simulink model "Controller"  (R2018b)
settings: configuration reference "control_config" (kept outside this file)
values from neighbouring files (symbols this model uses):
  CONTROL_EXPORT = Simulink.Parameter(CONTROL_EXPORT_VALUE)    [controller_model_init.m]
  CONTROL_PARAM = Simulink.Parameter(CONTROL_PARAM_VALUE)    [controller_model_init.m]
undefined symbols (not defined in the file or in its folder): actuator_cmd, CONTROL_CONST, ControlMode, DiscIntNeverNeededParam, PilotMode, timestamp, VehicleStatus, VTOLState
libraries: simulink x31, FMT_Model_Lib x20
(part 2 of 3)

== system Controller/Controller/VTOL_Control_Allocation/VTOL_Control_Allocation/VTOL1/actuator_cmd_routing ==
  cmd_in : Inport
  status : Inport  Port=2
  Disarm : Subsystem
  Multiport Switch : MultiPortSwitch  DataPortForDefault=Additional data port  DiagnosticForDefault=None
  Standby : Subsystem
  cmd_out : Outport
  wires:
  Multiport Switch/1 -> cmd_out/1
  status/1 -> Multiport Switch/1
  cmd_in/1 -> Multiport Switch/4
  Disarm/1(actuator_cmd) -> Multiport Switch/5, Multiport Switch/2
  Standby/1(actuator_cmd) -> Multiport Switch/3

== system Controller/Controller/VTOL_Control_Allocation/VTOL_Control_Allocation/VTOL2/FW_Control_Allocation ==
  fw_torque_cmd : Inport
  fw_force_cmd : Inport  Port=2
  FMS_Out : Inport  Port=3
  Bias : Bias  Bias=1500
  Bias1 : Bias  Bias=CONTROL_PARAM.SERVO1_BIAS
  Bias2 : Bias  Bias=CONTROL_PARAM.SERVO2_BIAS
  Bias3 : Bias  Bias=CONTROL_PARAM.SERVO3_BIAS
  Bias4 : Bias  Bias=CONTROL_PARAM.SERVO4_BIAS
  Data Type Conversion{,1..3} (4 alike) : DataTypeConversion  OutDataTypeStr=uint16
  Demux : Demux
  FW_Effective_Matrix : Subsystem
  Gain1 : Gain  Gain=[500;500;500;500]  OutDataTypeStr=Inherit: Same as input  ParamDataTypeStr=Inherit: Same as input
  Multiply1 : Product  Multiplication=Matrix(*)  OutDataTypeStr=Inherit: Same as first input
  Mux1 : Mux  Inputs=5
  Saturation1 : Saturate  UpperLimit=up_limit  LowerLimit=lo_limit  OutDataTypeStr=uint16
  Saturation4 : Saturate  UpperLimit=1  LowerLimit=0
  Saturation5 : Saturate  UpperLimit=1  LowerLimit=-1
  Selector : Selector  InputPortWidth=3  IndexOptions=Index vector (dialog)  Indices=1  OutputSizes=1
  Signal_Select : Subsystem  Commented=on
  fw_throttle_mapping : Subsystem
  fw_actuator_cmd : Outport
  wires:
  Demux/1 -> Bias1/1
  Gain1/1 -> Bias/1
  Saturation5/1 -> Multiply1/2
  Saturation4/1 -> fw_throttle_mapping/1(thrust_cmd)
  Selector/1 -> Saturation4/1
  Demux/2 -> Bias2/1
  Demux/4 -> Bias4/1
  FW_Effective_Matrix/1(EffecMat) -> Multiply1/1
  fw_force_cmd/1 -> Selector/1
  Demux/3 -> Bias3/1
  Mux1/1 -> Saturation1/1
  Multiply1/1 -> Gain1/1
  fw_torque_cmd/1 -> Saturation5/1
  fw_throttle_mapping/1(throttle_cmd) -> Mux1/1, Signal_Select/1(throttle_cmd_in)  "main_rotor"
  FMS_Out/1 -> Signal_Select/2(FMS_Out)
  Bias/1 -> Demux/1
  Saturation1/1 -> fw_actuator_cmd/1
  Bias1/1 -> Data Type Conversion/1
  Bias2/1 -> Data Type Conversion1/1
  Bias3/1 -> Data Type Conversion2/1
  Bias4/1 -> Data Type Conversion3/1
  Data Type Conversion/1 -> Mux1/2  "aileron_left"
  Data Type Conversion1/1 -> Mux1/3  "aileron_right"
  Data Type Conversion2/1 -> Mux1/4  "tail_left"
  Data Type Conversion3/1 -> Mux1/5  "tail_right"

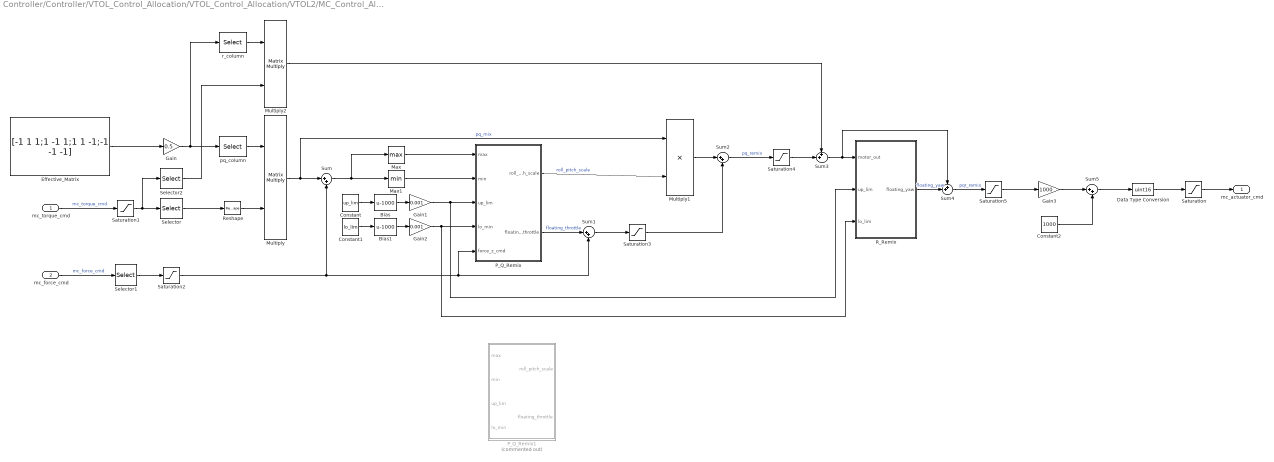
== system Controller/Controller/VTOL_Control_Allocation/VTOL_Control_Allocation/VTOL2/MC_Control_Allocation ==
  mc_torque_cmd : Inport
  mc_force_cmd : Inport  Port=2
  Bias : Bias  Bias=-1000
  Bias1 : Bias  Bias=-1000
  Constant : Constant  Value=up_lim  OutDataTypeStr=single
  Constant1 : Constant  Value=lo_lim  OutDataTypeStr=single
  Constant2 : Constant  Value=1000  OutDataTypeStr=uint32
  Data Type Conversion : DataTypeConversion  OutDataTypeStr=uint16
  Effective_Matrix : Constant  Value=[-1 1 1;1 -1 1;1 1 -1;-1 -1 -1]  OutDataTypeStr=single
  Gain : Gain  Gain=0.5
  Gain1 : Gain  Gain=0.001
  Gain2 : Gain  Gain=0.001
  Gain3 : Gain  Gain=1000  OutDataTypeStr=uint32
  Max : MinMax  Function=max
  Max1 : MinMax
  Multiply : Product  Multiplication=Matrix(*)  OutDataTypeStr=single
  Multiply1 : Product  OutDataTypeStr=single
  Multiply2 : Product  Multiplication=Matrix(*)  OutDataTypeStr=single
  P_Q_Remix : Subsystem
  P_Q_Remix1 : Subsystem  Commented=on
  R_Remix : MATLAB Function  TreatAsAtomicUnit=on
  Reshape : Reshape  OutputDimensionality=Column vector (2-D)
  Saturation : Saturate  UpperLimit=up_lim  LowerLimit=lo_lim
  Saturation1 : Saturate  UpperLimit=1  LowerLimit=-1
  Saturation{2..5} (4 alike) : Saturate  UpperLimit=1  LowerLimit=0
  Selector : Selector  InputPortWidth=3  IndexOptions=Index vector (dialog)  Indices=[1 2]  OutputSizes=1
  Selector1 : Selector  InputPortWidth=3  IndexOptions=Index vector (dialog)  Indices=3  OutputSizes=1
  Selector2 : Selector  InputPortWidth=3  IndexOptions=Index vector (dialog)  Indices=3  OutputSizes=1
  Sum{,1..2,5} (4 alike) : Sum  Inputs=|++
  Sum3 : Sum  Inputs=++|
  Sum4 : Sum  Inputs=++|
  pq_column : Selector  NumberOfDimensions=2  InputPortWidth=3  IndexOptions=Index vector (dialog),Index vector (dialog)  Indices=[1:4],[1 2]  OutputSizes=1,1
  r_column : Selector  NumberOfDimensions=2  InputPortWidth=3  IndexOptions=Index vector (dialog),Index vector (dialog)  Indices=[1:4],3  OutputSizes=1,1
  mc_actuator_cmd : Outport
  wires:
  Multiply/1 -> Multiply1/1, Sum/1  "pq_mix"
  Effective_Matrix/1 -> Gain/1
  mc_force_cmd/1 -> Selector1/1  "mc_force_cmd"
  Sum/1 -> Max/1, Max1/1
  Saturation/1 -> mc_actuator_cmd/1
  Reshape/1 -> Multiply/2
  Selector/1 -> Reshape/1
  Saturation1/1 -> Selector2/1, Selector/1
  Selector1/1 -> Saturation2/1
  pq_column/1 -> Multiply/1
  Max/1 -> P_Q_Remix/1(max)
  Max1/1 -> P_Q_Remix/2(min)
  Gain/1 -> r_column/1, pq_column/1
  P_Q_Remix/2(floating_throttle) -> Sum1/1  "floating_throttle"
  P_Q_Remix/1(roll_pitch_scale) -> Multiply1/2  "roll_pitch_scale"
  Multiply1/1 -> Sum2/1
  Sum1/1 -> Saturation3/1
  Sum2/1 -> Saturation4/1  "pq_remix"
  r_column/1 -> Multiply2/1
  Selector2/1 -> Multiply2/2
  Multiply2/1 -> Sum3/1
  Saturation4/1 -> Sum3/2
  Sum3/1 -> Sum4/1, R_Remix/1(motor_out)
  Constant/1 -> Bias/1
  Constant1/1 -> Bias1/1
  R_Remix/1(floating_yaw) -> Sum4/2  "floating_yaw"
  Sum4/1 -> Saturation5/1  "pqr_remix"
  Data Type Conversion/1 -> Saturation/1
  Bias/1 -> Gain1/1
  Gain1/1 -> R_Remix/2(up_lim), P_Q_Remix/3(up_lim)
  Bias1/1 -> Gain2/1
  Gain2/1 -> R_Remix/3(lo_lim), P_Q_Remix/4(lo_min)
  mc_torque_cmd/1 -> Saturation1/1  "mc_torque_cmd"
  Sum5/1 -> Data Type Conversion/1
  Saturation5/1 -> Gain3/1
  Gain3/1 -> Sum5/1
  Constant2/1 -> Sum5/2
  Saturation2/1 -> Sum1/2, P_Q_Remix/5(force_z_cmd), Sum/2
  Saturation3/1 -> Sum2/2

== system Controller/Controller/VTOL_Control_Allocation/VTOL_Control_Allocation/VTOL2/actuator_cmd_routing ==
  cmd_in : Inport
  status : Inport  Port=2
  Disarm : Subsystem
  Multiport Switch : MultiPortSwitch  DataPortForDefault=Additional data port  DiagnosticForDefault=None
  Standby : Subsystem
  cmd_out : Outport
  wires:
  Multiport Switch/1 -> cmd_out/1
  Standby/1(actuator_cmd) -> Multiport Switch/3
  status/1 -> Multiport Switch/1
  cmd_in/1 -> Multiport Switch/4
  Disarm/1(actuator_cmd) -> Multiport Switch/5, Multiport Switch/2

== system Controller/Controller/FW_Controller/FW_Controller/Attitude_Control/Innerloop_Rate_Control/PI_Control ==
  error : Inport
  reset : Inport  Port=2
  Add1 : Sum
  I_Control : Subsystem  mask{p_ki=CONTROL_PARAM.FW_ROLL_RATE_I, q_ki=CONTROL_PARAM.FW_PITCH_RATE_I, r_ki=CONTROL_PARAM.FW_YAW_RATE_I, max_i=CONTROL_PARAM.FW_RATE_I_MAX, min_i=CONTROL_PARAM.FW_RATE_I_MIN}
  P_Control : Subsystem  mask{p_kp=CONTROL_PARAM.FW_ROLL_RATE_P, q_kp=CONTROL_PARAM.FW_PITCH_RATE_P, r_kp=CONTROL_PARAM.FW_YAW_RATE_P}
  pi_out : Outport
  wires:
  Add1/1 -> pi_out/1
  I_Control/1(i_out) -> Add1/2  "fw_i_out"
  error/1 -> P_Control/1(err), I_Control/1(err)
  P_Control/1(p_out) -> Add1/1  "fw_p_out"
  reset/1 -> I_Control/2(reset)

== system Controller/Controller/FW_Controller/FW_Controller/Attitude_Control/Innerloop_Rate_Control/PI_scaler ==
  VT : Inport
  Divide : Product  Inputs=*/
  First Order LPF : FMT_Model_Lib/Filter/First Order LPF  fc=5
      settings: SourceProductName=FMT Toolbox
  Saturation : Saturate  UpperLimit=1  LowerLimit=0
  Square : Math  Operator=square  SaturateOnIntegerOverflow=on
  Square1 : Math  Operator=square  SaturateOnIntegerOverflow=on
  trim_speed : Constant  Value=CONTROL_PARAM.FW_AIRSPEED_TRIM
  PI_scale : Outport
  wires:
  Square1/1 -> Divide/2
  trim_speed/1 -> Square/1
  Square/1 -> Divide/1
  VT/1 -> Square1/1
  Saturation/1 -> First Order LPF/1
  Divide/1 -> Saturation/1
  First Order LPF/1 -> PI_scale/1

== system Controller/Controller/FW_Controller/FW_Controller/Attitude_Control/Innerloop_Rate_Control/VT_scaler ==
  VT : Inport
  Divide : Product  Inputs=*/
  First Order LPF : FMT_Model_Lib/Filter/First Order LPF  fc=5
      settings: SourceProductName=FMT Toolbox
  Saturation : Saturate  UpperLimit=1  LowerLimit=0
  trim_speed : Constant  Value=CONTROL_PARAM.FW_AIRSPEED_TRIM
  FF_scale : Outport
  wires:
  trim_speed/1 -> Divide/1
  VT/1 -> Divide/2
  Saturation/1 -> First Order LPF/1
  Divide/1 -> Saturation/1
  First Order LPF/1 -> FF_scale/1

== system Controller/Controller/FW_Controller/FW_Controller/Attitude_Control/Outloop_Angle_Control/Attitude_Controller ==
  att_cmd : Inport
  INS_Out : Inport  Port=2
  Error : Subsystem
  P_Controller : Subsystem
  phi_theta_rate_cmd : Outport
  wires:
  INS_Out/1 -> Error/2(INS_Out)
  P_Controller/1(u) -> phi_theta_rate_cmd/1
  att_cmd/1 -> Error/1(att_cmd)
  Error/1(euler_err_rad) -> P_Controller/1(error)

== system Controller/Controller/FW_Controller/FW_Controller/Attitude_Control/Outloop_Angle_Control/Heading_Controller ==
  fw_att_cmd : Inport
  FMS_Out : Inport  Port=2
  VT : Inport  Port=3
  Bus Selector2 : BusSelector  OutputSignals=psi_rate_cmd
  Demux : Demux  Outputs=2
  Saturation : Saturate  UpperLimit=CONTROL_PARAM.FW_R_CMD_LIM  LowerLimit=-CONTROL_PARAM.FW_R_CMD_LIM
  Sum : Sum  Inputs=++|
  Turning_Coordination : Subsystem
  psi_rate_cmd : Outport
  wires:
  Turning_Coordination/1(psi_rate_sp) -> Sum/2  "fw_psi_rate_sp"
  Sum/1 -> Saturation/1
  FMS_Out/1 -> Bus Selector2/1
  VT/1 -> Turning_Coordination/3(VT)
  Bus Selector2/1 -> Sum/1  "<psi_rate_cmd>"
  fw_att_cmd/1 -> Demux/1
  Demux/1 -> Turning_Coordination/1(phi_sp)
  Demux/2 -> Turning_Coordination/2(theta_sp)
  Saturation/1 -> psi_rate_cmd/1

== system Controller/Controller/FW_Controller/FW_Controller/Attitude_Control/Outloop_Angle_Control/Signal_Select ==
  att_cmd_rad : Inport
  FMS_Out : Inport  Port=2
  Bus Selector : BusSelector  OutputSignals=ctrl_mode
  Bus Selector1 : BusSelector  OutputSignals=phi_cmd
  Bus Selector2 : BusSelector  OutputSignals=ctrl_mode
  Bus Selector3 : BusSelector  OutputSignals=theta_cmd
  Compare To Constant : simulink/Logic and Bit Operations/Compare To Constant  relop===  const=uint8([ControlMode.Stabilize, ControlMode.ALTCTL])  OutDataTypeStr=boolean
  Compare To Constant1 : simulink/Logic and Bit Operations/Compare To Constant  relop===  const=uint8([ControlMode.Stabilize])  OutDataTypeStr=boolean
  Logical Operator : Logic  Operator=OR  Inputs=1  AllPortsSameDT=off  OutDataTypeStr=boolean
  Logical Operator1 : Logic  Operator=OR  Inputs=1  AllPortsSameDT=off  OutDataTypeStr=boolean
  Mux : Mux  Inputs=2
  Selector : Selector  InputPortWidth=2  IndexOptions=Index vector (dialog)  Indices=1  OutputSizes=1
  Selector1 : Selector  InputPortWidth=2  IndexOptions=Index vector (dialog)  Indices=2  OutputSizes=1
  Switch : Switch  Criteria=u2 > Threshold
  Switch1 : Switch  Criteria=u2 > Threshold
  fw_att_cmd : Outport
  wires:
  Compare To Constant/1 -> Logical Operator/1
  att_cmd_rad/1 -> Selector/1, Selector1/1
  Bus Selector/1 -> Compare To Constant/1  "<ctrl_mode>"
  FMS_Out/1 -> Bus Selector2/1, Bus Selector3/1, Bus Selector1/1, Bus Selector/1
  Bus Selector1/1 -> Switch/1  "<phi_cmd>"
  Logical Operator/1 -> Switch/2
  Selector/1 -> Switch/3
  Logical Operator1/1 -> Switch1/2
  Compare To Constant1/1 -> Logical Operator1/1
  Bus Selector2/1 -> Compare To Constant1/1  "<ctrl_mode>"
  Bus Selector3/1 -> Switch1/1  "<theta_cmd>"
  Selector1/1 -> Switch1/3
  Switch/1 -> Mux/1  "phi_cmd"
  Switch1/1 -> Mux/2  "theta_cmd"
  Mux/1 -> fw_att_cmd/1

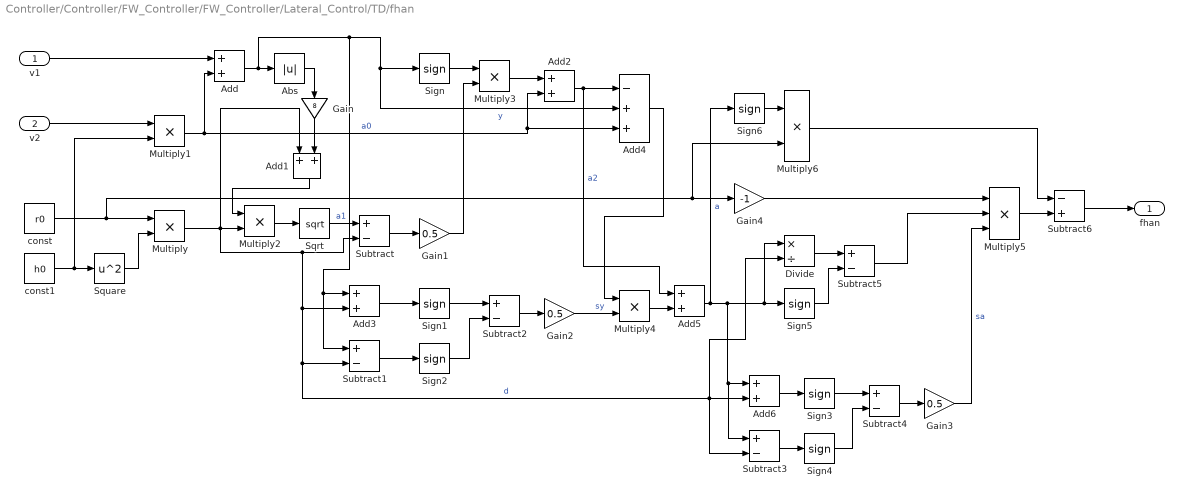
== system Controller/Controller/FW_Controller/FW_Controller/Lateral_Control/TD/fhan  ==
  v1 : Inport
  v2 : Inport  Port=2
  Abs : Abs
  Add{,1..3,5..6} (6 alike) : Sum  OutDataTypeStr=Inherit: Same as first input
  Add4 : Sum  Inputs=-++
  Divide : Product  Inputs=*/
  Gain : Gain  Gain=8
  Gain1 : Gain  Gain=0.5  OutDataTypeStr=Inherit: Same as input
  Gain2 : Gain  Gain=0.5  OutDataTypeStr=Inherit: Same as input
  Gain3 : Gain  Gain=0.5  OutDataTypeStr=Inherit: Same as input
  Gain4 : Gain  Gain=-1  OutDataTypeStr=Inherit: Same as input
  Multiply{,1..3} (4 alike) : Product  OutDataTypeStr=Inherit: Same as first input
  Multiply4 : Product  OutDataTypeStr=single
  Multiply5 : Product  Inputs=3
  Multiply6 : Product  OutDataTypeStr=single
  Sign{,1..6} (7 alike) : Signum
  Sqrt : Sqrt  SaturateOnIntegerOverflow=on
  Square : Math  Operator=square  SaturateOnIntegerOverflow=on
  Subtract{,1..5} (6 alike) : Sum  Inputs=+-  OutDataTypeStr=Inherit: Same as first input
  Subtract6 : Sum  Inputs=-+  OutDataTypeStr=Inherit: Same as first input
  const : Constant  Value=r0  OutDataTypeStr=single
  const1 : Constant  Value=h0  OutDataTypeStr=single
  fhan : Outport
  wires:
  v1/1 -> Add/1
  Sign/1 -> Multiply3/1
  Gain2/1 -> Multiply4/2  "sy"
  v2/1 -> Multiply1/1
  Gain3/1 -> Multiply5/3  "sa"
  Subtract/1 -> Gain1/1
  Subtract6/1 -> fhan/1
  Sign2/1 -> Subtract2/2
  Sign4/1 -> Subtract4/2
  Abs/1 -> Gain/1
  Add4/1 -> Multiply4/1
  Sign5/1 -> Subtract5/2
  Sqrt/1 -> Subtract/1  "a1"
  Subtract3/1 -> Sign4/1
  Add1/1 -> Multiply2/1
  Subtract1/1 -> Sign2/1
  Divide/1 -> Subtract5/1
  Multiply3/1 -> Add2/1
  Gain/1 -> Add1/2
  const/1 -> Multiply6/2, Gain4/1, Multiply/1
  Add3/1 -> Sign1/1
  Subtract5/1 -> Multiply5/2
  Multiply4/1 -> Add5/2
  const1/1 -> Multiply1/2, Square/1
  Add5/1 -> Sign6/1, Sign5/1, Divide/1, Subtract3/1, Add6/1  "a"
  Multiply1/1 -> Add4/3, Add2/2, Add/2  "a0"
  Add/1 -> Subtract1/1, Add3/1, Add4/2, Sign/1, Abs/1  "y"
  Subtract2/1 -> Gain2/1
  Add2/1 -> Add4/1, Add5/1  "a2"
  Subtract4/1 -> Gain3/1
  Gain4/1 -> Multiply5/1
  Multiply5/1 -> Subtract6/2
  Sign6/1 -> Multiply6/1
  Sign3/1 -> Subtract4/1
  Add6/1 -> Sign3/1
  Multiply/1 -> Subtract/2, Divide/2, Subtract3/2, Add6/2, Subtract1/2, Add3/2, Add1/1, Multiply2/2  "d"
  Multiply6/1 -> Subtract6/1
  Gain1/1 -> Multiply3/2
  Square/1 -> Multiply/2
  Multiply2/1 -> Sqrt/1
  Sign1/1 -> Subtract2/1

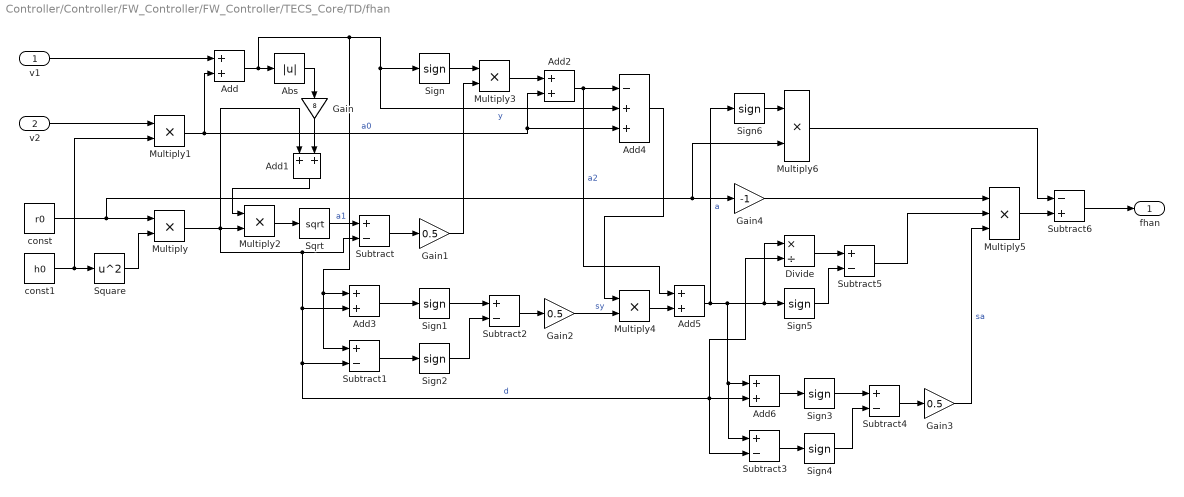
== system Controller/Controller/FW_Controller/FW_Controller/TECS_Core/TD/fhan  ==
  v1 : Inport
  v2 : Inport  Port=2
  Abs : Abs
  Add{,1..3,5..6} (6 alike) : Sum  OutDataTypeStr=Inherit: Same as first input
  Add4 : Sum  Inputs=-++
  Divide : Product  Inputs=*/
  Gain : Gain  Gain=8
  Gain1 : Gain  Gain=0.5  OutDataTypeStr=Inherit: Same as input
  Gain2 : Gain  Gain=0.5  OutDataTypeStr=Inherit: Same as input
  Gain3 : Gain  Gain=0.5  OutDataTypeStr=Inherit: Same as input
  Gain4 : Gain  Gain=-1  OutDataTypeStr=Inherit: Same as input
  Multiply{,1..3} (4 alike) : Product  OutDataTypeStr=Inherit: Same as first input
  Multiply4 : Product  OutDataTypeStr=single
  Multiply5 : Product  Inputs=3
  Multiply6 : Product  OutDataTypeStr=single
  Sign{,1..6} (7 alike) : Signum
  Sqrt : Sqrt  SaturateOnIntegerOverflow=on
  Square : Math  Operator=square  SaturateOnIntegerOverflow=on
  Subtract{,1..5} (6 alike) : Sum  Inputs=+-  OutDataTypeStr=Inherit: Same as first input
  Subtract6 : Sum  Inputs=-+  OutDataTypeStr=Inherit: Same as first input
  const : Constant  Value=r0  OutDataTypeStr=single
  const1 : Constant  Value=h0  OutDataTypeStr=single
  fhan : Outport
  wires:
  v1/1 -> Add/1
  Sign/1 -> Multiply3/1
  Gain2/1 -> Multiply4/2  "sy"
  v2/1 -> Multiply1/1
  Gain3/1 -> Multiply5/3  "sa"
  Subtract/1 -> Gain1/1
  Subtract6/1 -> fhan/1
  Sign2/1 -> Subtract2/2
  Sign4/1 -> Subtract4/2
  Abs/1 -> Gain/1
  Add4/1 -> Multiply4/1
  Sign5/1 -> Subtract5/2
  Sqrt/1 -> Subtract/1  "a1"
  Subtract3/1 -> Sign4/1
  Add1/1 -> Multiply2/1
  Subtract1/1 -> Sign2/1
  Divide/1 -> Subtract5/1
  Multiply3/1 -> Add2/1
  Gain/1 -> Add1/2
  const/1 -> Multiply6/2, Gain4/1, Multiply/1
  Add3/1 -> Sign1/1
  Subtract5/1 -> Multiply5/2
  Multiply4/1 -> Add5/2
  const1/1 -> Multiply1/2, Square/1
  Add5/1 -> Sign6/1, Sign5/1, Divide/1, Subtract3/1, Add6/1  "a"
  Multiply1/1 -> Add4/3, Add2/2, Add/2  "a0"
  Add/1 -> Subtract1/1, Add3/1, Add4/2, Sign/1, Abs/1  "y"
  Subtract2/1 -> Gain2/1
  Add2/1 -> Add4/1, Add5/1  "a2"
  Subtract4/1 -> Gain3/1
  Gain4/1 -> Multiply5/1
  Multiply5/1 -> Subtract6/2
  Sign6/1 -> Multiply6/1
  Sign3/1 -> Subtract4/1
  Add6/1 -> Sign3/1
  Multiply/1 -> Subtract/2, Divide/2, Subtract3/2, Add6/2, Subtract1/2, Add3/2, Add1/1, Multiply2/2  "d"
  Multiply6/1 -> Subtract6/1
  Gain1/1 -> Multiply3/2
  Square/1 -> Multiply/2
  Multiply2/1 -> Sqrt/1
  Sign1/1 -> Subtract2/1

== system Controller/Controller/FW_Controller/FW_Controller/TECS_Core/path_angle_control/Flight_Path_Angle ==
  INS_Out : Inport
  gamma_dir : Inport  Port=2
  speed : Inport  Port=3
  Asin : Trigonometry  Operator=atan
  Bus Selector2 : BusSelector  OutputSignals=vd
  Dead Zone : DeadZone  LowerValue=-0.1  UpperValue=0.1  SaturateOnIntegerOverflow=on
  Divide : Product  Inputs=/*
  Gain : Gain  Gain=-1
  Multiply1 : Product
  Saturation1 : Saturate  UpperLimit=pi/4  LowerLimit=-pi/4
  gamma : Outport
  wires:
  INS_Out/1 -> Bus Selector2/1
  Gain/1 -> Divide/2
  Divide/1 -> Asin/1
  Bus Selector2/1 -> Dead Zone/1  "<vd>"
  Asin/1 -> Multiply1/2
  speed/1 -> Divide/1
  Saturation1/1 -> gamma/1
  Dead Zone/1 -> Gain/1
  Multiply1/1 -> Saturation1/1
  gamma_dir/1 -> Multiply1/1

== system Controller/Controller/FW_Controller/FW_Controller/TECS_Core/path_angle_control/Fly_Speed ==
  INS_Out : Inport
  Bitwise AND : simulink/Logic and Bit Operations/Bitwise Operator  logicop=AND  UseBitMask=on  BitMask=bin2dec('10000')  BitMaskRealWorld=Stored Integer
  Bus Selector1 : BusSelector  OutputSignals=flag,airspeed
  Bus Selector2 : BusSelector  OutputSignals=vn,ve,vd
  Bus Selector3 : BusSelector  OutputSignals=quat
  Multiply : Product  Multiplication=Matrix(*)
  Mux : Mux  Inputs=3
  Quaternion To DCM : FMT_Model_Lib/Quaternion/Quaternion To DCM
      settings: SourceProductName=FMT Toolbox
  Saturation : Saturate  UpperLimit=100  LowerLimit=8
  Selector : Selector  InputPortWidth=3  IndexOptions=Index vector (dialog)  Indices=1  OutputSizes=1
  Switch : Switch  Criteria=u2 > Threshold
  speed : Outport
  wires:
  Bus Selector3/1 -> Quaternion To DCM/1  "<quat>"
  Multiply/1 -> Selector/1
  Bus Selector2/3 -> Mux/3  "<vd>"
  Mux/1 -> Multiply/2
  Quaternion To DCM/1 -> Multiply/1
  Bus Selector2/2 -> Mux/2  "<ve>"
  Bus Selector2/1 -> Mux/1  "<vn>"
  Bus Selector1/2 -> Switch/3  "<airspeed>"
  Bus Selector1/1 -> Bitwise AND/1  "<flag>"
  Bitwise AND/1 -> Switch/2
  INS_Out/1 -> Bus Selector3/1, Bus Selector1/1, Bus Selector2/1
  Selector/1 -> Switch/1
  Switch/1 -> Saturation/1
  Saturation/1 -> speed/1

== system Controller/Controller/FW_Controller/FW_Controller/TECS_Core/path_angle_control/Subsystem ==
  INS_Out : Inport
  Bitwise AND : simulink/Logic and Bit Operations/Bitwise Operator  logicop=AND  UseBitMask=on  BitMask=bin2dec('10000')  BitMaskRealWorld=Stored Integer
  Bus Selector1 : BusSelector  OutputSignals=flag
  Bus Selector2 : BusSelector  OutputSignals=vn,ve,vd
  Bus Selector3 : BusSelector  OutputSignals=psi
  Constant : Constant  OutDataTypeStr=single
  Dead Zone : DeadZone  LowerValue=-1  UpperValue=1  SaturateOnIntegerOverflow=on
  Multiply : Product  Multiplication=Matrix(*)
  Mux : Mux  Inputs=3
  Psi To DCM : FMT_Model_Lib/Transformation/Psi To DCM
      settings: SourceProductName=FMT Toolbox
  Selector : Selector  InputPortWidth=3  IndexOptions=Index vector (dialog)  Indices=1  OutputSizes=1
  Sign : Signum
  Switch : Switch  Criteria=u2 > Threshold
  gamma_dir : Outport
  wires:
  Psi To DCM/1 -> Multiply/1
  Bus Selector2/3 -> Mux/3  "<vd>"
  Selector/1 -> Dead Zone/1
  Bus Selector2/2 -> Mux/2  "<ve>"
  Bus Selector3/1 -> Psi To DCM/1  "<psi>"
  Multiply/1 -> Selector/1
  Dead Zone/1 -> Sign/1
  Bus Selector2/1 -> Mux/1  "<vn>"
  Mux/1 -> Multiply/2
  INS_Out/1 -> Bus Selector1/1, Bus Selector2/1, Bus Selector3/1
  Sign/1 -> Switch/1
  Bus Selector1/1 -> Bitwise AND/1  "<flag>"
  Bitwise AND/1 -> Switch/2
  Switch/1 -> gamma_dir/1
  Constant/1 -> Switch/3

== system Controller/Controller/FW_Controller/FW_Controller/TECS_Core/path_angle_control/Target_Flight_Path_Angle ==
  FMS_Out : Inport
  gamma_dir : Inport  Port=2
  speed : Inport  Port=3
  Asin : Trigonometry  Operator=atan
  Bus Selector : BusSelector  OutputSignals=w_cmd
  Divide : Product  Inputs=*/
  Gain : Gain  Gain=-1
  Multiply1 : Product
  Saturation2 : Saturate  UpperLimit=pi/4  LowerLimit=-pi/4
  gamma_sp : Outport
  wires:
  FMS_Out/1 -> Bus Selector/1
  Bus Selector/1 -> Gain/1  "<w_cmd>"
  Divide/1 -> Asin/1
  Gain/1 -> Divide/1
  speed/1 -> Divide/2
  Saturation2/1 -> gamma_sp/1
  Asin/1 -> Multiply1/1
  Multiply1/1 -> Saturation2/1
  gamma_dir/1 -> Multiply1/2

== system Controller/Controller/FW_Controller/FW_Controller/TECS_Core/pitch_controller/D_control ==
  err : Inport
  reset : Inport  Port=2
  DT Filter : FMT_Model_Lib/Filter/DT Filter  fc=10
      settings: SourceProductName=FMT Toolbox
  Gain : Gain  Gain=CONTROL_PARAM.FW_TECS_PITCH_D
  d_out : Outport
  wires:
  reset/1 -> DT Filter/2
  DT Filter/1 -> Gain/1
  Gain/1 -> d_out/1
  err/1 -> DT Filter/1

== system Controller/Controller/FW_Controller/FW_Controller/TECS_Core/pitch_controller/I_control ==
  err : Inport
  reset : Inport  Port=2
  " " : DiscreteIntegrator  ExternalReset=level  InitialConditionSource=external  SampleTime=-1  LimitOutput=on  UpperSaturationLimit=CONTROL_PARAM.FW_TECS_PITCH_I_LIM  LowerSaturationLimit=-CONTROL_PARAM.FW_TECS_PITCH_I_LIM  ICPrevOutput=DiscIntNeverNeededParam  ICPrevScaledInput=DiscIntNeverNeededParam
  Gain3 : Gain  Gain=CONTROL_PARAM.FW_TECS_PITCH_I
  Zero1 : Constant  Value=0  OutDataTypeStr=Inherit: Inherit via back propagation
  i_out : Outport
  wires:
  Zero1/1 -> " "/3
  " "/1 -> i_out/1
  Gain3/1 -> " "/1
  err/1 -> Gain3/1
  reset/1 -> " "/2

== system Controller/Controller/MC_Controller/Horizontal_Control/Attitude_Controller/Inner_Loop/ATT_Cmd_Mixer ==
  FMS_Out : Inport
  euler_rate_cmd : Inport  Port=2
  aux_mc_cmd : Inport  Port=3
  INS_Out : Inport  Port=4
  Backward_Mixer : Subsystem  mask{max=8, min=2}
  Bus Selector1 : BusSelector  OutputSignals=ext_state
  Bus Selector2 : BusSelector  OutputSignals=psi_rate_cmd
  Bus Selector3 : BusSelector  OutputSignals=phi,theta
  Demux : Demux  Outputs=3
  Euler To Angle Rate : FMT_Model_Lib/Math/Euler To Angle Rate
      settings: SourceProductName=FMT Toolbox
  Fly_Speed : Subsystem
  Forward_Mixer : Subsystem  mask{max=8, min=2}
  Multiport Switch : MultiPortSwitch  DataPortOrder=Specify indices  DataPortIndices={uint8(VTOLState.ForwardTrans),uint8(VTOLState.BackwardTrans),uint8(VTOLState.Fixwing),uint8(VTOLState.Stall),uint8(VTOLState.Multicopter)}  DiagnosticForDefault=None
  Mux : Mux  Inputs=3
  Mux1 : Mux  Inputs=2
  Mux2 : Mux  Inputs=2
  Saturation : Saturate  UpperLimit=CONTROL_PARAM.MC_R_CMD_LIM  LowerLimit=-CONTROL_PARAM.MC_R_CMD_LIM
  Saturation1 : Saturate  UpperLimit=CONTROL_PARAM.MC_P_Q_CMD_LIM  LowerLimit=-CONTROL_PARAM.MC_P_Q_CMD_LIM
  Saturation2 : Saturate  UpperLimit=CONTROL_PARAM.MC_P_Q_CMD_LIM  LowerLimit=-CONTROL_PARAM.MC_P_Q_CMD_LIM
  rate_cmd_radPs : Outport
  wires:
  Bus Selector3/1 -> Mux2/1  "<phi>"
  Mux2/1 -> Euler To Angle Rate/1
  Bus Selector3/2 -> Mux2/2  "<theta>"
  Bus Selector2/1 -> Mux1/2  "<psi_rate_cmd>"
  FMS_Out/1 -> Bus Selector2/1, Bus Selector1/1
  INS_Out/1 -> Fly_Speed/1(INS_Out), Bus Selector3/1
  Euler To Angle Rate/1 -> Demux/1  "ang_rate"
  euler_rate_cmd/1 -> Mux1/1
  Demux/1 -> Saturation1/1
  Demux/2 -> Saturation2/1
  Demux/3 -> Saturation/1
  Saturation1/1 -> Mux/1
  Mux/1 -> rate_cmd_radPs/1
  Saturation2/1 -> Mux/2
  Saturation/1 -> Mux/3
  Bus Selector1/1 -> Multiport Switch/1  "<ext_state>"
  Multiport Switch/1 -> Euler To Angle Rate/2  "euler_rate"
  aux_mc_cmd/1 -> Multiport Switch/5, Multiport Switch/4, Forward_Mixer/2(aux_cmd), Backward_Mixer/2(aux_cmd)  "aux_rate_cmd"
  Backward_Mixer/1(mix_rate_cmd) -> Multiport Switch/3
  Forward_Mixer/1(mix_rate_cmd) -> Multiport Switch/2
  Mux1/1 -> Forward_Mixer/1(mc_cmd), Backward_Mixer/1(mc_cmd), Multiport Switch/6  "mc_rate_cmd"
  Fly_Speed/1(speed) -> Backward_Mixer/3(VT), Forward_Mixer/3(VT)

== system Controller/Controller/MC_Controller/Horizontal_Control/Attitude_Controller/Inner_Loop/Rate_Controller ==
  rate_cmd_radPs : Inport
  INS_Out : Inport  Port=2
  reset : Inport  Port=3
  Error : Subsystem
  Feedforward_Controller : Subsystem
  PID_Controller : Subsystem
  Sum : Sum  Inputs=++|
  rate_dot_cmd_B : Outport
  wires:
  INS_Out/1 -> Error/2(INS_Out)
  Error/1(rate_err_radPs) -> PID_Controller/1(rate_err_radPs)
  rate_cmd_radPs/1 -> Feedforward_Controller/1(rate_cmd_radPs), Error/1(rate_cmd_radPs)  "yy1"
  reset/1 -> PID_Controller/2(reset)
  PID_Controller/1(rate_dot_cmd_B) -> Sum/2
  Feedforward_Controller/1(rate_dot_cmd_B) -> Sum/1
  Sum/1 -> rate_dot_cmd_B/1

== system Controller/Controller/MC_Controller/Horizontal_Control/Attitude_Controller/Outter_Loop/Attitude_Controller ==
  att_cmd_rad : Inport
  INS_Out : Inport  Port=2
  Error : Subsystem
  Sqrt_Root_Controller : Subsystem
  euler_rate_cmd_radPs : Outport
  wires:
  INS_Out/1 -> Error/2(INS_Out)
  Sqrt_Root_Controller/1(euler_rate_cmd_radPs) -> euler_rate_cmd_radPs/1
  att_cmd_rad/1 -> Error/1(att_cmd)
  Error/1(euler_err_rad) -> Sqrt_Root_Controller/1(euler_err_rad)

== system Controller/Controller/MC_Controller/Horizontal_Control/Attitude_Controller/Outter_Loop/Signal_Select ==
  note: mode:
      | 0: Unknown
      | 1: Mission
      | 2: Position
      | 3: Altitude Hold
      | 4: Manual Mode
      | 5: Acro Mode
      | 6: Offboard
  att_cmd_rad : Inport
  FMS_Out : Inport  Port=2
  Bus Selector : BusSelector  OutputSignals=ctrl_mode
  Bus Selector1 : BusSelector  OutputSignals=phi_cmd,theta_cmd
  Compare To Constant : simulink/Logic and Bit Operations/Compare To Constant  relop===  const=uint8([ControlMode.Stabilize, ControlMode.ALTCTL])  OutDataTypeStr=boolean
  Compare To Constant1 : simulink/Logic and Bit Operations/Compare To Constant  relop===  const=uint8(ControlMode.Offboard)  OutDataTypeStr=boolean
  Logical Operator : Logic  Operator=OR  Inputs=1  AllPortsSameDT=off  OutDataTypeStr=boolean
  Mux : Mux  Inputs=2
  Offboard_Signal_Select : Subsystem
  Switch : Switch  Criteria=u2 > Threshold
  Switch1 : Switch  Criteria=u2 > Threshold
  out : Outport
  wires:
  Compare To Constant/1 -> Logical Operator/1
  Bus Selector1/2 -> Mux/2  "<theta_cmd>"
  Bus Selector1/1 -> Mux/1  "<phi_cmd>"
  Bus Selector/1 -> Compare To Constant1/1, Compare To Constant/1  "<ctrl_mode>"
  FMS_Out/1 -> Bus Selector/1, Bus Selector1/1, Offboard_Signal_Select/1(FMS_Out)
  Mux/1 -> Switch/1
  Switch/1 -> out/1
  Logical Operator/1 -> Switch/2
  Switch1/1 -> Switch/3
  Compare To Constant1/1 -> Switch1/2
  Offboard_Signal_Select/1(att_cmd_rad) -> Switch1/1
  att_cmd_rad/1 -> Offboard_Signal_Select/2(att_cmd_in), Switch1/3

== system Controller/Controller/MC_Controller/Horizontal_Control/Velocity_Controller/Error/Bus_Select ==
  INS_Out : Inport
  Bus Selector1 : BusSelector  OutputSignals=vn,ve
  Bus Selector2 : BusSelector  OutputSignals=psi
  Constant : Constant  Value=0  OutDataTypeStr=single
  Multiply : Product  Multiplication=Matrix(*)
  Mux2 : Mux  Inputs=3
  Psi To DCM : FMT_Model_Lib/Transformation/Psi To DCM
      settings: SourceProductName=FMT Toolbox
  Selector : Selector  InputPortWidth=3  IndexOptions=Index vector (dialog)  Indices=[1 2]  OutputSizes=1
  uv_est_C_mPs : Outport
  wires:
  Psi To DCM/1 -> Multiply/1
  Bus Selector2/1 -> Psi To DCM/1  "<psi>"
  Constant/1 -> Mux2/3  "<velD>"
  Mux2/1 -> Multiply/2
  Bus Selector1/2 -> Mux2/2  "<ve>"
  Bus Selector1/1 -> Mux2/1  "<vn>"
  INS_Out/1 -> Bus Selector2/1, Bus Selector1/1
  Multiply/1 -> Selector/1
  Selector/1 -> uv_est_C_mPs/1

== system Controller/Controller/MC_Controller/Horizontal_Control/Velocity_Controller/Error/TD ==
  v : Inport
  v0 : Inport  Port=2
  Integrator : DiscreteIntegrator  SampleTime=-1  ICPrevOutput=DiscIntNeverNeededParam  ICPrevScaledInput=DiscIntNeverNeededParam
  Integrator1 : DiscreteIntegrator  InitialConditionSource=external  SampleTime=-1  ICPrevOutput=DiscIntNeverNeededParam  ICPrevScaledInput=DiscIntNeverNeededParam
  Subtract : Sum  Inputs=+-
  "fhan " : Subsystem  mask{r0=6*9.806, h0=0.05}
      mask DialogControl ParameterGroupVar Prompt: fhan(v1,v2,r0,h0)
  v1 : Outport
  wires:
  Integrator1/1 -> Subtract/1, v1/1
  v/1 -> Subtract/2
  Integrator/1 -> "fhan "/2(v2), Integrator1/1  "v2"
  Subtract/1 -> "fhan "/1(v1)
  "fhan "/1(fhan) -> Integrator/1
  v0/1 -> Integrator1/2

== system Controller/Controller/MC_Controller/Horizontal_Control/Velocity_Controller/PID_Controller/D_Control ==
  err : Inport
  reset : Inport  Port=2
  DT Filter : FMT_Model_Lib/Filter/DT Filter  fc=10
      settings: SourceProductName=FMT Toolbox
  Multiply : Product  OutDataTypeStr=Inherit: Same as first input
  Saturation : Saturate  UpperLimit=max_d  LowerLimit=min_d
  kd : Constant  Value=kd  OutDataTypeStr=single
  d_out : Outport
  wires:
  err/1 -> DT Filter/1
  kd/1 -> Multiply/1
  Multiply/1 -> Saturation/1
  Saturation/1 -> d_out/1
  reset/1 -> DT Filter/2
  DT Filter/1 -> Multiply/2

== system Controller/Controller/MC_Controller/Horizontal_Control/Velocity_Controller/PID_Controller/I_Control ==
  err : Inport
  reset : Inport  Port=2
  Constant : Constant  Value=0  OutDataTypeStr=single
  Discrete-Time Integrator : DiscreteIntegrator  ExternalReset=level  InitialConditionSource=external  SampleTime=-1  LimitOutput=on  UpperSaturationLimit=max_i  LowerSaturationLimit=min_i  ICPrevOutput=DiscIntNeverNeededParam  ICPrevScaledInput=DiscIntNeverNeededParam
  Multiply : Product  OutDataTypeStr=Inherit: Same as first input
  ki : Constant  Value=ki  OutDataTypeStr=single
  i_out : Outport
  wires:
  err/1 -> Multiply/2
  Multiply/1 -> Discrete-Time Integrator/1
  reset/1 -> Discrete-Time Integrator/2
  Constant/1 -> Discrete-Time Integrator/3
  Discrete-Time Integrator/1 -> i_out/1
  ki/1 -> Multiply/1

== system Controller/Controller/MC_Controller/Horizontal_Control/Velocity_Controller/PID_Controller/P_Control ==
  err : Inport
  Multiply : Product  OutDataTypeStr=Inherit: Same as first input
  kp : Constant  Value=kp  OutDataTypeStr=single
  p_out : Outport
  wires:
  err/1 -> Multiply/2
  kp/1 -> Multiply/1
  Multiply/1 -> p_out/1

== system Controller/Controller/MC_Controller/Horizontal_Control/Velocity_Controller/Signal_Select/Offboard_Signal_Select ==
  FMS_Out : Inport
  acc_cmd_in : Inport  Port=2
  Bus Selector1 : BusSelector  OutputSignals=cmd_mask
  Bus Selector2 : BusSelector  OutputSignals=ax_cmd,ay_cmd
  Compare To Zero : simulink/Logic and Bit Operations/Compare To Zero  relop=>  OutDataTypeStr=boolean
  Compare To Zero2 : simulink/Logic and Bit Operations/Compare To Zero  relop=>  OutDataTypeStr=boolean
  Multiply2 : Product
  Multiply3 : Product
  Mux : Mux  Inputs=2
  Mux1 : Mux  Inputs=2
  Mux2 : Mux  Inputs=2
  Sum1 : Sum  Inputs=|++
  cmd_ax valid : simulink/Logic and Bit Operations/Bitwise Operator  logicop=AND  UseBitMask=on  BitMask=bin2dec('1000000000')  BitMaskRealWorld=Stored Integer
  cmd_ay valid : simulink/Logic and Bit Operations/Bitwise Operator  logicop=AND  UseBitMask=on  BitMask=bin2dec('10000000000')  BitMaskRealWorld=Stored Integer
  cmd_u valid : simulink/Logic and Bit Operations/Bitwise Operator  logicop=AND  UseBitMask=on  BitMask=bin2dec('1000000')  BitMaskRealWorld=Stored Integer
  cmd_v valid : simulink/Logic and Bit Operations/Bitwise Operator  logicop=AND  UseBitMask=on  BitMask=bin2dec('10000000')  BitMaskRealWorld=Stored Integer
  acc_cmd : Outport
  wires:
  Multiply2/1 -> Sum1/2
  FMS_Out/1 -> Bus Selector2/1, Bus Selector1/1
  Bus Selector1/1 -> cmd_v valid/1, cmd_u valid/1, cmd_ay valid/1, cmd_ax valid/1  "<cmd_mask>"
  Multiply3/1 -> Sum1/1
  cmd_u valid/1 -> Mux1/1
  cmd_v valid/1 -> Mux1/2
  Mux1/1 -> Compare To Zero/1
  acc_cmd_in/1 -> Multiply2/2
  Compare To Zero/1 -> Multiply2/1
  Bus Selector2/1 -> Mux/1  "<ax_cmd>"
  cmd_ax valid/1 -> Mux2/1
  cmd_ay valid/1 -> Mux2/2
  Mux2/1 -> Compare To Zero2/1
  Compare To Zero2/1 -> Multiply3/2
  Bus Selector2/2 -> Mux/2  "<ay_cmd>"
  Mux/1 -> Multiply3/1
  Sum1/1 -> acc_cmd/1

== system Controller/Controller/MC_Controller/Vertical_Control/Veloxity_Z_Controller/Error/TD ==
  v : Inport
  Integrator : DiscreteIntegrator  SampleTime=-1  ICPrevOutput=DiscIntNeverNeededParam  ICPrevScaledInput=DiscIntNeverNeededParam
  Integrator1 : DiscreteIntegrator  SampleTime=-1  ICPrevOutput=DiscIntNeverNeededParam  ICPrevScaledInput=DiscIntNeverNeededParam
  Subtract : Sum  Inputs=+-
  "fhan " : Subsystem  mask{r0=8*9.806, h0=0.05}
      mask DialogControl ParameterGroupVar Prompt: fhan(v1,v2,r0,h0)
  v1 : Outport
  wires:
  Integrator1/1 -> v1/1, Subtract/1
  v/1 -> Subtract/2
  Integrator/1 -> "fhan "/2(v2), Integrator1/1  "v2"
  Subtract/1 -> "fhan "/1(v1)
  "fhan "/1(fhan) -> Integrator/1

== system Controller/Controller/MC_Controller/Vertical_Control/Veloxity_Z_Controller/PID_Controller/D_Control ==
  err : Inport
  reset : Inport  Port=2
  DT Filter : FMT_Model_Lib/Filter/DT Filter  fc=10
      settings: SourceProductName=FMT Toolbox
  Multiply : Product  OutDataTypeStr=Inherit: Same as first input
  Saturation : Saturate  UpperLimit=max_d  LowerLimit=min_d
  kd : Constant  Value=kd  OutDataTypeStr=single
  d_out : Outport
  wires:
  err/1 -> DT Filter/1
  kd/1 -> Multiply/1
  Multiply/1 -> Saturation/1
  Saturation/1 -> d_out/1
  reset/1 -> DT Filter/2
  DT Filter/1 -> Multiply/2

== system Controller/Controller/MC_Controller/Vertical_Control/Veloxity_Z_Controller/PID_Controller/I_Control ==
  err : Inport
  slow_start : Inport  Port=2
  reset : Inport  Port=3
  Constant : Constant  Value=min_i  OutDataTypeStr=single
  Constant1 : Constant  Value=0  OutDataTypeStr=single
  Discrete-Time Integrator : DiscreteIntegrator  ExternalReset=level  InitialConditionSource=external  SampleTime=-1  LimitOutput=on  UpperSaturationLimit=max_i  LowerSaturationLimit=min_i  ICPrevOutput=DiscIntNeverNeededParam  ICPrevScaledInput=DiscIntNeverNeededParam
  Multiply : Product  OutDataTypeStr=Inherit: Same as first input
  Switch : Switch  Criteria=u2 > Threshold
  ki : Constant  Value=ki  OutDataTypeStr=single
  i_out : Outport
  wires:
  err/1 -> Multiply/2
  Multiply/1 -> Discrete-Time Integrator/1
  reset/1 -> Discrete-Time Integrator/2
  Discrete-Time Integrator/1 -> i_out/1
  ki/1 -> Multiply/1
  Constant/1 -> Switch/1
  Constant1/1 -> Switch/3
  Switch/1 -> Discrete-Time Integrator/3
  slow_start/1 -> Switch/2

== system Controller/Controller/MC_Controller/Vertical_Control/Veloxity_Z_Controller/PID_Controller/P_Control ==
  err : Inport
  Multiply : Product  OutDataTypeStr=Inherit: Same as first input
  kp : Constant  Value=kp  OutDataTypeStr=single
  p_out : Outport
  wires:
  err/1 -> Multiply/2
  kp/1 -> Multiply/1
  Multiply/1 -> p_out/1

== system Controller/Controller/VTOL_Control_Allocation/VTOL_Control_Allocation/VTOL1/FW_Control_Allocation/FW_Effective_Matrix ==
  Constant1 : Constant  Value=CONTROL_PARAM.FW_ROLL_EFFC*CONTROL_PARAM.FW_AILERON1_DIR  OutDataTypeStr=single
  Constant{3..6,8..11} (8 alike) : Constant  Value=0  OutDataTypeStr=single
  Constant12 : Constant  Value=CONTROL_PARAM.FW_YAW_EFFC*CONTROL_PARAM.FW_RUDDER_DIR  OutDataTypeStr=single
  Constant2 : Constant  Value=CONTROL_PARAM.FW_ROLL_EFFC*CONTROL_PARAM.FW_AILERON2_DIR  OutDataTypeStr=single
  Constant7 : Constant  Value=CONTROL_PARAM.FW_PITCH_EFFC*CONTROL_PARAM.FW_ELEVATOR_DIR  OutDataTypeStr=single
  Matrix Concatenate : Concatenate  NumInputs=3  Mode=Multidimensional array  ConcatenateDimension=2
  Vector Concatenate : Concatenate  NumInputs=4
  Vector Concatenate1 : Concatenate  NumInputs=4
  Vector Concatenate2 : Concatenate  NumInputs=4
  EffecMat : Outport
  wires:
  Constant7/1 -> Vector Concatenate1/3
  Constant8/1 -> Vector Concatenate1/4
  Constant9/1 -> Vector Concatenate2/1
  Constant12/1 -> Vector Concatenate2/4
  Constant3/1 -> Vector Concatenate/3
  Vector Concatenate/1 -> Matrix Concatenate/1
  Matrix Concatenate/1 -> EffecMat/1
  Constant2/1 -> Vector Concatenate/2
  Constant11/1 -> Vector Concatenate2/3
  Constant10/1 -> Vector Concatenate2/2
  Constant1/1 -> Vector Concatenate/1
  Vector Concatenate2/1 -> Matrix Concatenate/3
  Constant4/1 -> Vector Concatenate/4
  Vector Concatenate1/1 -> Matrix Concatenate/2
  Constant5/1 -> Vector Concatenate1/1
  Constant6/1 -> Vector Concatenate1/2

== system Controller/Controller/VTOL_Control_Allocation/VTOL_Control_Allocation/VTOL1/FW_Control_Allocation/Signal_Select ==
  throttle_cmd_in : Inport
  FMS_Out : Inport  Port=2
  Bus Selector1 : BusSelector  OutputSignals=throttle_cmd,ctrl_mode
  Compare To Constant : simulink/Logic and Bit Operations/Compare To Constant  relop=<=  const=uint8(ControlMode.Stabilize)  OutDataTypeStr=boolean
  Switch : Switch  Criteria=u2 > Threshold
  throttle_cmd : Outport
  wires:
  Compare To Constant/1 -> Switch/2
  throttle_cmd_in/1 -> Switch/3  "ff6"
  Bus Selector1/2 -> Compare To Constant/1  "<ctrl_mode>"
  Bus Selector1/1 -> Switch/1  "<throttle_cmd>"
  FMS_Out/1 -> Bus Selector1/1
  Switch/1 -> throttle_cmd/1

== system Controller/Controller/VTOL_Control_Allocation/VTOL_Control_Allocation/VTOL1/FW_Control_Allocation/fw_throttle_mapping ==
  thrust_cmd : Inport
  Constant1 : Constant  Value=1000  OutDataTypeStr=uint32
  Data Type Conversion : DataTypeConversion  OutDataTypeStr=uint16
  Gain1 : Gain  Gain=1000  OutDataTypeStr=uint32
  Sum1 : Sum  Inputs=|++
  throttle_cmd : Outport
  wires:
  Sum1/1 -> Data Type Conversion/1
  thrust_cmd/1 -> Gain1/1
  Data Type Conversion/1 -> throttle_cmd/1
  Constant1/1 -> Sum1/2
  Gain1/1 -> Sum1/1

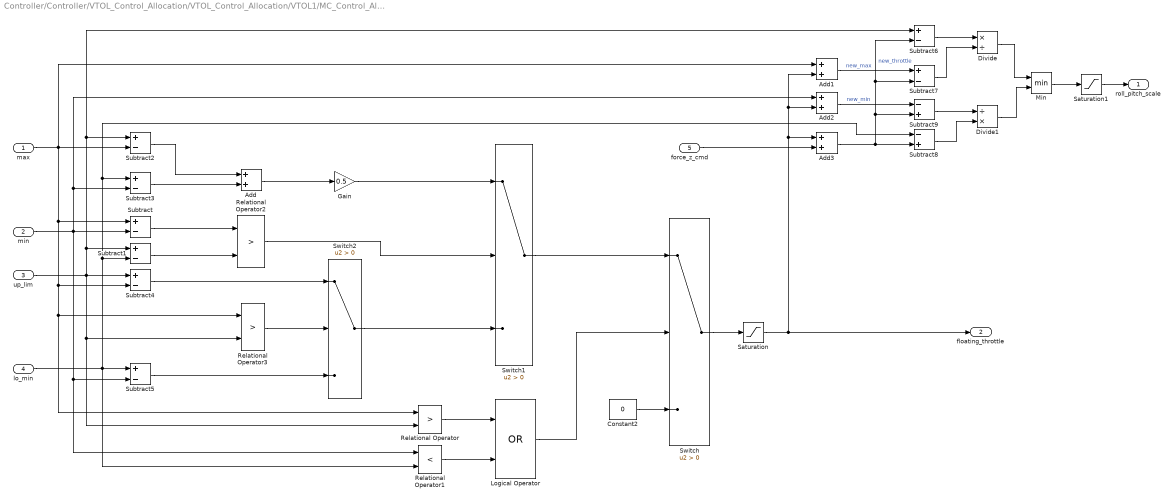
== system Controller/Controller/VTOL_Control_Allocation/VTOL_Control_Allocation/VTOL1/MC_Control_Allocation/P_Q_Remix ==
  max : Inport
  min : Inport  Port=2
  up_lim : Inport  Port=3
  lo_min : Inport  Port=4
  force_z_cmd : Inport  Port=5
  Add{,1..3} (4 alike) : Sum
  Constant2 : Constant  Value=0  OutDataTypeStr=single
  Divide : Product  Inputs=*/
  Divide1 : Product  Inputs=/*
  Gain : Gain  Gain=0.5
  Logical Operator : Logic  Operator=OR  AllPortsSameDT=off  OutDataTypeStr=boolean
  Min : MinMax  Inputs=2
  Relational Operator : RelationalOperator  Operator=>  OutDataTypeStr=boolean  RndMeth=Simplest
  Relational Operator1 : RelationalOperator  Operator=<  OutDataTypeStr=boolean  RndMeth=Simplest
  Relational Operator2 : RelationalOperator  Operator=>  OutDataTypeStr=boolean  RndMeth=Simplest
  Relational Operator3 : RelationalOperator  Operator=>  OutDataTypeStr=boolean  RndMeth=Simplest
  Saturation : Saturate  UpperLimit=0.2  LowerLimit=-0.2
  Saturation1 : Saturate  UpperLimit=1  LowerLimit=0.5
  Subtract{,1..7} (8 alike) : Sum  Inputs=+-
  Subtract8 : Sum  Inputs=-+
  Subtract9 : Sum  Inputs=-+
  Switch : Switch  Criteria=u2 > Threshold
  Switch1 : Switch  Criteria=u2 > Threshold
  Switch2 : Switch  Criteria=u2 > Threshold
  roll_pitch_scale : Outport
  floating_throttle : Outport  Port=2
  wires:
  max/1 -> Subtract/1, Relational Operator3/1, Relational Operator/1, Subtract4/2, Add1/1, Subtract2/2
  up_lim/1 -> Relational Operator/2, Relational Operator3/2, Subtract6/1, Subtract2/1, Subtract1/1, Subtract4/1
  min/1 -> Add2/1, Subtract3/2, Subtract/2, Relational Operator1/1, Subtract5/2
  lo_min/1 -> Subtract8/1, Subtract3/1, Subtract1/2, Relational Operator1/2, Subtract5/1
  Relational Operator/1 -> Logical Operator/1
  Relational Operator1/1 -> Logical Operator/2
  Logical Operator/1 -> Switch/2
  Constant2/1 -> Switch/3
  Subtract/1 -> Relational Operator2/1
  Subtract1/1 -> Relational Operator2/2
  Relational Operator2/1 -> Switch1/2
  Subtract2/1 -> Add/1
  Subtract3/1 -> Add/2
  Add/1 -> Gain/1
  Gain/1 -> Switch1/1
  Relational Operator3/1 -> Switch2/2
  Subtract4/1 -> Switch2/1
  Switch1/1 -> Switch/1
  Switch2/1 -> Switch1/3
  Subtract5/1 -> Switch2/3
  Switch/1 -> Saturation/1
  force_z_cmd/1 -> Add3/2
  Add1/1 -> Subtract7/1  "new_max"
  Add2/1 -> Subtract9/1  "new_min"
  Add3/1 -> Subtract7/2, Subtract6/2, Subtract9/2, Subtract8/2  "new_throttle"
  Subtract6/1 -> Divide/1
  Subtract7/1 -> Divide/2
  Subtract8/1 -> Divide1/2
  Subtract9/1 -> Divide1/1
  Divide/1 -> Min/1
  Divide1/1 -> Min/2
  Min/1 -> Saturation1/1
  Saturation1/1 -> roll_pitch_scale/1
  Saturation/1 -> Add3/1, Add2/2, Add1/2, floating_throttle/1

== system Controller/Controller/VTOL_Control_Allocation/VTOL_Control_Allocation/VTOL1/actuator_cmd_routing/Disarm ==
  Bias : Bias  Bias=CONTROL_PARAM.SERVO1_BIAS
  Bias1 : Bias  Bias=CONTROL_PARAM.SERVO2_BIAS
  Bias2 : Bias  Bias=CONTROL_PARAM.SERVO3_BIAS
  Bias3 : Bias  Bias=CONTROL_PARAM.SERVO4_BIAS
  Constant : Constant  Value=1500  OutDataTypeStr=single
  Data Type Conversion : DataTypeConversion  OutDataTypeStr=uint16
  Disarm : Constant  Value=[1000 1000 1000 1000 1000]'  VectorParams1D=off  OutDataTypeStr=single
  Mux : Mux  Inputs=5
  Reshape : Reshape  OutputDimensionality=Column vector (2-D)
  Saturation : Saturate  UpperLimit=2000  LowerLimit=1000
  actuator_cmd : Outport
  wires:
  Disarm/1 -> Mux/1
  Constant/1 -> Bias3/1, Bias2/1, Bias1/1, Bias/1
  Mux/1 -> Reshape/1
  Data Type Conversion/1 -> actuator_cmd/1
  Saturation/1 -> Data Type Conversion/1
  Reshape/1 -> Saturation/1
  Bias/1 -> Mux/2
  Bias1/1 -> Mux/3
  Bias2/1 -> Mux/4
  Bias3/1 -> Mux/5

== system Controller/Controller/VTOL_Control_Allocation/VTOL_Control_Allocation/VTOL1/actuator_cmd_routing/Standby ==
  Bias : Bias  Bias=CONTROL_PARAM.SERVO1_BIAS
  Bias1 : Bias  Bias=CONTROL_PARAM.SERVO2_BIAS
  Bias2 : Bias  Bias=CONTROL_PARAM.SERVO3_BIAS
  Bias3 : Bias  Bias=CONTROL_PARAM.SERVO4_BIAS
  Constant : Constant  Value=1500  OutDataTypeStr=single
  Data Type Conversion : DataTypeConversion  OutDataTypeStr=uint16
  Mux : Mux  Inputs=5
  Reshape : Reshape  OutputDimensionality=Column vector (2-D)
  Saturation : Saturate  UpperLimit=2000  LowerLimit=1000
  Standby : Constant  Value=[1150 1150 1150 1150 1000]'  VectorParams1D=off  OutDataTypeStr=single
  actuator_cmd : Outport
  wires:
  Bias3/1 -> Mux/5
  Bias2/1 -> Mux/4
  Bias1/1 -> Mux/3
  Bias/1 -> Mux/2
  Reshape/1 -> Saturation/1
  Saturation/1 -> Data Type Conversion/1
  Mux/1 -> Reshape/1
  Constant/1 -> Bias/1, Bias1/1, Bias2/1, Bias3/1
  Standby/1 -> Mux/1
  Data Type Conversion/1 -> actuator_cmd/1

== system Controller/Controller/VTOL_Control_Allocation/VTOL_Control_Allocation/VTOL2/FW_Control_Allocation/FW_Effective_Matrix ==
  Constant1 : Constant  Value=CONTROL_PARAM.FW_ROLL_EFFC*CONTROL_PARAM.FW_AILERON1_DIR  OutDataTypeStr=single
  Constant{3..6,9..10} (6 alike) : Constant  Value=0  OutDataTypeStr=single
  Constant11 : Constant  Value=CONTROL_PARAM.FW_YAW_EFFC*CONTROL_PARAM.FW_TAIL1_DIR  OutDataTypeStr=single
  Constant12 : Constant  Value=CONTROL_PARAM.FW_YAW_EFFC*CONTROL_PARAM.FW_TAIL2_DIR  OutDataTypeStr=single
  Constant2 : Constant  Value=CONTROL_PARAM.FW_ROLL_EFFC*CONTROL_PARAM.FW_AILERON2_DIR  OutDataTypeStr=single
  Constant7 : Constant  Value=CONTROL_PARAM.FW_PITCH_EFFC*CONTROL_PARAM.FW_TAIL1_DIR  OutDataTypeStr=single
  Constant8 : Constant  Value=-CONTROL_PARAM.FW_PITCH_EFFC*CONTROL_PARAM.FW_TAIL2_DIR  OutDataTypeStr=single
  Matrix Concatenate : Concatenate  NumInputs=3  Mode=Multidimensional array  ConcatenateDimension=2
  Vector Concatenate : Concatenate  NumInputs=4
  Vector Concatenate1 : Concatenate  NumInputs=4
  Vector Concatenate2 : Concatenate  NumInputs=4
  EffecMat : Outport
  wires:
  Constant7/1 -> Vector Concatenate1/3
  Constant8/1 -> Vector Concatenate1/4
  Constant9/1 -> Vector Concatenate2/1
  Constant12/1 -> Vector Concatenate2/4
  Constant3/1 -> Vector Concatenate/3
  Vector Concatenate/1 -> Matrix Concatenate/1
  Matrix Concatenate/1 -> EffecMat/1
  Constant2/1 -> Vector Concatenate/2
  Constant11/1 -> Vector Concatenate2/3
  Constant10/1 -> Vector Concatenate2/2
  Constant1/1 -> Vector Concatenate/1
  Vector Concatenate2/1 -> Matrix Concatenate/3
  Constant4/1 -> Vector Concatenate/4
  Vector Concatenate1/1 -> Matrix Concatenate/2
  Constant5/1 -> Vector Concatenate1/1
  Constant6/1 -> Vector Concatenate1/2

== system Controller/Controller/VTOL_Control_Allocation/VTOL_Control_Allocation/VTOL2/FW_Control_Allocation/Signal_Select ==
  throttle_cmd_in : Inport
  FMS_Out : Inport  Port=2
  Bus Selector1 : BusSelector  OutputSignals=throttle_cmd,ctrl_mode
  Compare To Constant : simulink/Logic and Bit Operations/Compare To Constant  relop=<=  const=uint8(ControlMode.Stabilize)  OutDataTypeStr=boolean
  Switch : Switch  Criteria=u2 > Threshold
  throttle_cmd : Outport
  wires:
  Compare To Constant/1 -> Switch/2
  throttle_cmd_in/1 -> Switch/3  "ff6"
  Bus Selector1/2 -> Compare To Constant/1  "<ctrl_mode>"
  Bus Selector1/1 -> Switch/1  "<throttle_cmd>"
  FMS_Out/1 -> Bus Selector1/1
  Switch/1 -> throttle_cmd/1

== system Controller/Controller/VTOL_Control_Allocation/VTOL_Control_Allocation/VTOL2/FW_Control_Allocation/fw_throttle_mapping ==
  thrust_cmd : Inport
  Constant1 : Constant  Value=1000  OutDataTypeStr=uint32
  Data Type Conversion : DataTypeConversion  OutDataTypeStr=uint16
  Gain1 : Gain  Gain=1000  OutDataTypeStr=uint32
  Sum1 : Sum  Inputs=|++
  throttle_cmd : Outport
  wires:
  Sum1/1 -> Data Type Conversion/1
  thrust_cmd/1 -> Gain1/1
  Data Type Conversion/1 -> throttle_cmd/1
  Constant1/1 -> Sum1/2
  Gain1/1 -> Sum1/1

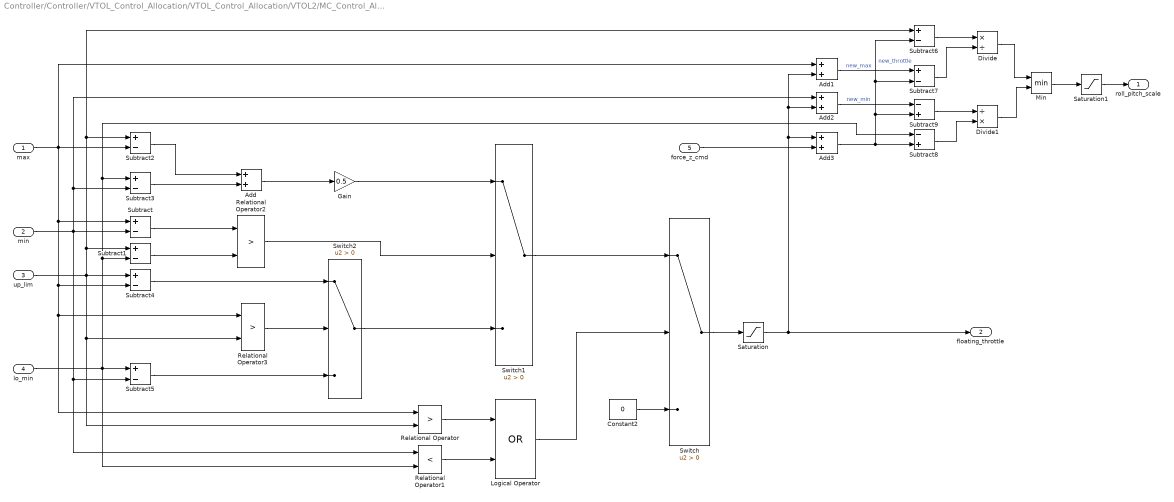
== system Controller/Controller/VTOL_Control_Allocation/VTOL_Control_Allocation/VTOL2/MC_Control_Allocation/P_Q_Remix ==
  max : Inport
  min : Inport  Port=2
  up_lim : Inport  Port=3
  lo_min : Inport  Port=4
  force_z_cmd : Inport  Port=5
  Add{,1..3} (4 alike) : Sum
  Constant2 : Constant  Value=0  OutDataTypeStr=single
  Divide : Product  Inputs=*/
  Divide1 : Product  Inputs=/*
  Gain : Gain  Gain=0.5
  Logical Operator : Logic  Operator=OR  AllPortsSameDT=off  OutDataTypeStr=boolean
  Min : MinMax  Inputs=2
  Relational Operator : RelationalOperator  Operator=>  OutDataTypeStr=boolean  RndMeth=Simplest
  Relational Operator1 : RelationalOperator  Operator=<  OutDataTypeStr=boolean  RndMeth=Simplest
  Relational Operator2 : RelationalOperator  Operator=>  OutDataTypeStr=boolean  RndMeth=Simplest
  Relational Operator3 : RelationalOperator  Operator=>  OutDataTypeStr=boolean  RndMeth=Simplest
  Saturation : Saturate  UpperLimit=0.2  LowerLimit=-0.2
  Saturation1 : Saturate  UpperLimit=1  LowerLimit=0.5
  Subtract{,1..7} (8 alike) : Sum  Inputs=+-
  Subtract8 : Sum  Inputs=-+
  Subtract9 : Sum  Inputs=-+
  Switch : Switch  Criteria=u2 > Threshold
  Switch1 : Switch  Criteria=u2 > Threshold
  Switch2 : Switch  Criteria=u2 > Threshold
  roll_pitch_scale : Outport
  floating_throttle : Outport  Port=2
  wires:
  max/1 -> Subtract/1, Relational Operator3/1, Relational Operator/1, Subtract4/2, Add1/1, Subtract2/2
  up_lim/1 -> Relational Operator/2, Relational Operator3/2, Subtract6/1, Subtract2/1, Subtract1/1, Subtract4/1
  min/1 -> Add2/1, Subtract3/2, Subtract/2, Relational Operator1/1, Subtract5/2
  lo_min/1 -> Subtract8/1, Subtract3/1, Subtract1/2, Relational Operator1/2, Subtract5/1
  Relational Operator/1 -> Logical Operator/1
  Relational Operator1/1 -> Logical Operator/2
  Logical Operator/1 -> Switch/2
  Constant2/1 -> Switch/3
  Subtract/1 -> Relational Operator2/1
  Subtract1/1 -> Relational Operator2/2
  Relational Operator2/1 -> Switch1/2
  Subtract2/1 -> Add/1
  Subtract3/1 -> Add/2
  Add/1 -> Gain/1
  Gain/1 -> Switch1/1
  Relational Operator3/1 -> Switch2/2
  Subtract4/1 -> Switch2/1
  Switch1/1 -> Switch/1
  Switch2/1 -> Switch1/3
  Subtract5/1 -> Switch2/3
  Switch/1 -> Saturation/1
  force_z_cmd/1 -> Add3/2
  Add1/1 -> Subtract7/1  "new_max"
  Add2/1 -> Subtract9/1  "new_min"
  Add3/1 -> Subtract7/2, Subtract6/2, Subtract9/2, Subtract8/2  "new_throttle"
  Subtract6/1 -> Divide/1
  Subtract7/1 -> Divide/2
  Subtract8/1 -> Divide1/2
  Subtract9/1 -> Divide1/1
  Divide/1 -> Min/1
  Divide1/1 -> Min/2
  Min/1 -> Saturation1/1
  Saturation1/1 -> roll_pitch_scale/1
  Saturation/1 -> Add3/1, Add2/2, Add1/2, floating_throttle/1
